simulink model "advanced_active_clamping"  (R2023b)
settings: Solver=ode1be  StartTime=0.0  StopTime=simlength  FixedStep=tc  RelTol=1e-3
values from neighbouring files (symbols this model uses):
  Rgate = 2.5    [init_model.m]
  Rgate_internal = 4    [init_model.m]
  t0_dpt = 5e-6    (= 5e-06)    [init_model.m]
  t1_dpt = t0_dpt + delta_time_first_pulse    (= 0.000105)    [init_model.m]
  t2_dpt = t1_dpt + deadtime    (= 0.000108)    [init_model.m]
  t3_dpt = t2_dpt + delta_time_discharge    (= 0.000128)    [init_model.m]
  t4_dpt = t3_dpt + deadtime    (= 0.000131)    [init_model.m]
  t5_dpt = t4_dpt + delta_time_second_pulse    (= 0.000166)    [init_model.m]
  t6_dpt = t5_dpt + deadtime    (= 0.000169)    [init_model.m]
  Vdc = 1400    [init_model.m]
  Vgate_h = 15    [init_model.m]
  Vgate_l = -7    [init_model.m]
libraries: fl_lib x55, nesl_utility x11, ee_lib x10, simulink x4
(part 3 of 3)

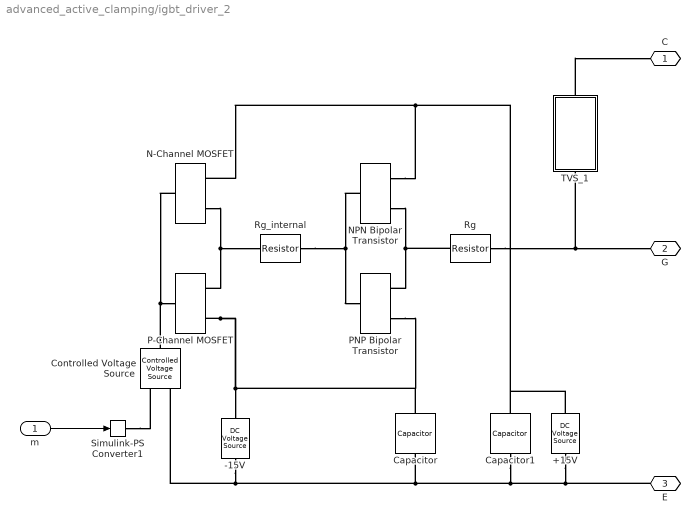
== system advanced_active_clamping/igbt_driver_2 ==
  m : Inport
  +15V : fl_lib/Electrical/Electrical Sources/DC Voltage Source  v0=15 V
  -15V : fl_lib/Electrical/Electrical Sources/DC Voltage Source  v0=-15 V
  Capacitor : fl_lib/Electrical/Electrical Elements/Capacitor  c=100e-9 F  r=1e-6 Ohm  g=0 1/Ohm  i_specify=off  i_priority=None  i=0 A  i_nominal_specify=off  i_nominal_unit=A  i_nominal_value=1  v_specify=off  v_priority=None  v=0 V  v_nominal_specify=off  v_nominal_unit=V  v_nominal_value=1  vc_specify=off  vc_priority=High  vc=0 V  vc_nominal_specify=off  vc_nominal_unit=V  vc_nominal_value=1
  Capacitor1 : fl_lib/Electrical/Electrical Elements/Capacitor  c=100e-9 F  r=1e-6 Ohm  g=0 1/Ohm  i_specify=off  i_priority=None  i=0 A  i_nominal_specify=off  i_nominal_unit=A  i_nominal_value=1  v_specify=off  v_priority=None  v=0 V  v_nominal_specify=off  v_nominal_unit=V  v_nominal_value=1  vc_specify=off  vc_priority=High  vc=0 V  vc_nominal_specify=off  vc_nominal_unit=V  vc_nominal_value=1
  Controlled Voltage Source : fl_lib/Electrical/Electrical Sources/Controlled Voltage Source
  N-Channel MOSFET : ee_lib/Semiconductors & Converters/N-Channel MOSFET  paramTerminal=ee.enum.mosfet.numberOfTerminals.three  parameterization=ee.enum.mosfet.parameterization.datasheet  Beta=5.0 A/V^2  Rds=0.025 Ohm  Id=100e-3 A  Vgs=10 V  Vth=1.7 V  Vth0=1.7 V  lam=0 1/V  gamma_vth=0.5 V^(1/2)  phib=0.5 V  Vth1=1.9071 V  Vbs1=-1 V  Vth2=2.066 V  Vbs2=-2 V  Tmeas=25 degC  Vgs_vec=[-1, -.5, 2, 3, 4, 5] V  Vds_vec=[0, 2, 4, 8, 12, 16, 20] V  Vbs_vec=[0, -4, -6, -12] V  T_vec=[25, 125] degC  Vth_vec=[.4, 1.2, 1.4, 1.45] V  Vth_mat=[.4, .35; 1.2, 1.15; 1.4, 1.35; 1.45, 1.4] V  Ids_mat=[0, 0, 0, 0, 0, 0, 0; 0, 0, 0, 0, 0, 0, 0; 0, .003, .0038, .0043, .0046, .0048, .0049; 0, .0055, .008, .009, .0095, .01, .0101; 0, .0115, .016, .018, .019, .0195, .02; 0, .0152, .0225, .0265, .028, .0295, .03] A  Ids_mat0=[0, 0, 0, 0, 0, 0, 0; 0, 0, 0, 0, 0, 0, 0; 0, .003, .0038, .0043, .0046, .0048, .0049; 0, .0055, .008, .009, .0095, .01, .0101; 0, .0115, .016, .018, .019, .0195, .02; 0, .0152, .0225, .0265, .028, .0295, .03] A  Ids_mat_3D=zeros(6, 7, 2) A  Ids_mat_3D0=zeros(6, 7, 2) A  IV_table_symmetry=ee.enum.mosfet.symmetricNIV.no  RS=0.0001 Ohm  RD=0.01 Ohm  RB=0.001 Ohm  C_param=ee.enum.mosfet.capacitanceParam.fixedciss  C_GS=270 pF  C_GD=80 pF  C_GB=0 pF  C_DS=0 pF  C_iss=350 pF  C_rss=80 pF  C_oss=0 pF  C_iss_vec=[720, 700, 590, 470, 390, 310] pF  C_rss_vec=[450, 400, 300, 190, 95, 55] pF  C_oss_vec=[900, 810, 690, 420, 270, 170] pF  C_GS_vec=[270, 300, 290, 280, 295, 255] pF  C_GD_vec=[450, 400, 300, 190, 95, 55] pF  C_GB_vec=[270, 300, 290, 280, 295, 255] pF  C_Vgs_vec=0 V  C_DS_vec=[450, 410, 390, 230, 175, 115] pF  C_Vds_vec=[.1, .3, 1, 3, 10, 30] V  V_GS_for_cap_data=0 V  charge_linearity_param=ee.enum.mosfet.cgdLinearity.constant  C_OX=200 pF  V_C_OX=-0.5 V  charge_linearity_param_vgb=ee.enum.mosfet.cgbLinearity.instantly  charge_linearity_param_with_vgb=ee.enum.mosfet.cgbLinearityWithSeparateCgb.instantly  Di_param=ee.enum.mosfet.diodeParam.no  IsDiode=1e-12 A  Vbi=0.6 V  n=1  Cj0Diode=0 pF  TT=50e-9 s  Tmeas_dio=25 degC  TableTypeNoT=ee.enum.mosfet.tableType.IfMat  TableType=ee.enum.diode.tableType.IfMat  IfVec=[.07, .12, .19, 1.75, 4.24, 7.32, 11.2] A  IfMat=[.07, .12, .19, 1.75, 4.24, 7.32, 11.2; .16, .3, .72, 2.14, 4.02, 6.35, 9.12] A  VfVecV=[.9, 1.15, 1.25, 1.5, 1.75, 2.17, 2.6, 2.85] V  VfMatV=[.9, 1.15, 1.25, 1.5, 1.75, 2.17, 2.6, 2.85; .58, .68, .75, 1.1, 1.38, 1.77, 2.27, 2.7] V  TjVec=[25, 125] degC  VfVec=[.5, .7, .9, 1.3, 1.7, 2.1, 2.5] V  IfVecV=[.1, .2, .5, 1, 2, 4, 7, 10] A  prmDatasheet=ee.enum.temperatureParameterization.none  prmEquCoeff=ee.enum.temperatureParameterization.none  dVth_dT=-6 mV/K  dVth0_dT=-6 mV/K  Rds_T2=0.037 Ohm  BEXDatasheet=-1.5  BEXEquCoeff=-1.5  etaisDatasheet=3  etaisEquCoeff=3  Tmeas2=125 degC  etaisTabulated=3  TdeviceDatasheet=25 degC  TdeviceEquCoeff=25 degC  TdeviceTabulated=25 degC  enable_faults=simscape.enum.onoff.off  fault_trigger=ee.enum.faults.faultTrigger.temporal  t_fault=inf s  max_permissible_Vgs=inf V  max_permissible_Vds=inf V  max_permissible_Vdb=inf V  max_permissible_Ids=inf A  t_fail_on_Ids=1 s  max_permissible_Idiode=inf A  t_fail_on_Idiode=1 s  max_permissible_dVdt=inf V/s  tau_fault=1e-3 s  fault_types=ee.enum.mosfet.faults.open  fault_types_4T=ee.enum.mosfet.faultsFourTerminals.open  RG_open=1e6 Ohm  RD_open=1000 Ohm  RS_open=1000 Ohm  RB_open=1000 Ohm  GDS_short=1000 1/Ohm  GDB_short=1000 1/Ohm  GSB_short=1000 1/Ohm  location_GOS=0  G_GOS=1000 1/Ohm  D_GOS=ee.enum.include.no  Is_GOS=0 A  Vbi_GOS=0.6 V  n_GOS=1  Cj0_GOS=0 pF  TT_GOS=50e-9 s  Beta_scale=100  dVth_faulted=0 V  lam_faulted=0 1/V  gamma_scale=100  dPhib_faulted=0 V  Vgs_vec_faulted=[-1, -.5, 2, 3, 4, 5] V  Vds_vec_faulted=[0, 2, 4, 8, 12, 16, 20] V  Vbs_vec_faulted=[0, -4, -6, -12] V  Vth_vec_faulted=[.4, 1.2, 1.4, 1.45] V  Vth_mat_faulted=[.4, .35; 1.2, 1.15; 1.4, 1.35; 1.45, 1.4] V  Ids_mat_faulted=[0, 0, 0, 0, 0, 0, 0; 0, 0, 0, 0, 0, 0, 0; 0, .003, .0038, .0043, .0046, .0048, .0049; 0, .0055, .008, .009, .0095, .01, .0101; 0, .0115, .016, .018, .019, .0195, .02; 0, .0152, .0225, .0265, .028, .0295, .03] A  Ids_mat0_faulted=[0, 0, 0, 0, 0, 0, 0; 0, 0, 0, 0, 0, 0, 0; 0, .003, .0038, .0043, .0046, .0048, .0049; 0, .0055, .008, .009, .0095, .01, .0101; 0, .0115, .016, .018, .019, .0195, .02; 0, .0152, .0225, .0265, .028, .0295, .03] A  Ids_mat_3D_faulted=zeros(6, 7, 2) A  Ids_mat_3D0_faulted=zeros(6, 7, 2) A  RS_faulted=0.0001 Ohm  RD_faulted=0.01 Ohm  RB_faulted=0.001 Ohm  IsDiode_faulted=0 A  Vbi_faulted=0.6 V  n_faulted=1  Cj0Diode_scale=100  TT_faulted=50e-9 s  IfVec_faulted=[.07, .12, .19, 1.75, 4.24, 7.32, 11.2] A  IfMat_faulted=[.07, .12, .19, 1.75, 4.24, 7.32, 11.2; .16, .3, .72, 2.14, 4.02, 6.35, 9.12] A  VfVecV_faulted=[.9, 1.15, 1.25, 1.5, 1.75, 2.17, 2.6, 2.85] V  VfMatV_faulted=[.9, 1.15, 1.25, 1.5, 1.75, 2.17, 2.6, 2.85; .58, .68, .75, 1.1, 1.38, 1.77, 2.27, 2.7] V  VfVec_faulted=[.5, .7, .9, 1.3, 1.7, 2.1, 2.5] V  IfVecV_faulted=[.1, .2, .5, 1, 2, 4, 7, 10] A  C_GS_scale=100  C_GD_scale=100  C_GB_scale=100  C_DS_scale=100  C_OX_scale=100  V_C_OX_faulted=-0.5 V  C_iss_vec_faulted=[720, 700, 590, 470, 390, 310] pF  C_rss_vec_faulted=[450, 400, 300, 190, 95, 55] pF  C_oss_vec_faulted=[900, 810, 690, 420, 270, 170] pF  C_GS_vec_faulted=[270, 300, 290, 280, 295, 255] pF  C_GD_vec_faulted=[450, 400, 300, 190, 95, 55] pF  C_GB_vec_faulted=[270, 300, 290, 280, 295, 255] pF  C_Vgs_vec_faulted=0 V  C_DS_vec_faulted=[450, 410, 390, 230, 175, 115] pF  C_Vds_vec_faulted=[.1, .3, 1, 3, 10, 30] V  V_GS_for_cap_data_faulted=0 V  i_g_specify=off  i_g_priority=None  i_g=0 A  i_g_nominal_specify=off  i_g_nominal_unit=A  i_g_nominal_value=1  i_d_specify=off  i_d_priority=None  i_d=0 A  i_d_nominal_specify=off  i_d_nominal_unit=A  i_d_nominal_value=1  i_b_specify=off  i_b_priority=None  i_b=0 A  i_b_nominal_specify=off  i_b_nominal_unit=A  i_b_nominal_value=1  voltage_gs_specify=off  voltage_gs_priority=None  voltage_gs=0 V  voltage_gs_nominal_specify=off  voltage_gs_nominal_unit=V  voltage_gs_nominal_value=1  voltage_ds_specify=off  voltage_ds_priority=None  voltage_ds=0 V  voltage_ds_nominal_specify=off  voltage_ds_nominal_unit=V  voltage_ds_nominal_value=1  voltage_bs_specify=off  voltage_bs_priority=None  voltage_bs=0 V  voltage_bs_nominal_specify=off  voltage_bs_nominal_unit=V  voltage_bs_nominal_value=1  v_Cgs_specify=off  v_Cgs_priority=High  v_Cgs=0 V  v_Cgs_nominal_specify=off  v_Cgs_nominal_unit=V  v_Cgs_nominal_value=1  v_Cds_specify=off  v_Cds_priority=High  v_Cds=0 V  v_Cds_nominal_specify=off  v_Cds_nominal_unit=V  v_Cds_nominal_value=1  v_Cbs_specify=off  v_Cbs_priority=High  v_Cbs=0 V  v_Cbs_nominal_specify=off  v_Cbs_nominal_unit=V  v_Cbs_nominal_value=1  faulted_specify=off  faulted_priority=None  faulted=0  faulted_nominal_specify=off  faulted_nominal_unit=1  faulted_nominal_value=1  thermal_network_parameterization=ee.enum.thermalNetworkTopology.junctionCase  Rth=[0, 10] K/W  Rth_Cauer=[1, 3, 10] K/W  Rth_Foster=[4, 6] K/W  thermal_mass_parameterization=ee.enum.thermalNetwork.timeconstant  thermal_mass=[0, 1] J/K  thermal_mass_Cauer=[.1, .3, 1] J/K  thermal_mass_Foster=[1.5, 3] J/K  thermal_time_constant=[0, 10] s  thermal_time_constant_Cauer=[1, 3, 10] s  thermal_time_constant_Foster=[6, 18] s  thermal_mass_initial_temperatures=[25, 25] degC  thermal_mass_initial_temperatures_Cauer=[25, 25, 25] degC  Tvec_initial_Foster=[25, 25, 25, 25] degC  max_permissible_temperature=inf K  t_fail_on_temperature=1 s  betaref=18 A/V^2  Vfbref=-1.1 V  gamma=3.5 V^(1/2)  phib2ref=1 V  thesatref=0.4 1/V  alpha=0  Vp=5e-2 V  thesrref=0 1/V  m=8  Tref=25 degC  Rsref=2e-3 Ohm  Rdref=0.17 Ohm  Rgref=8.4 Ohm  Rbref=2e-3 Ohm  Cox=1500 pF  Cgso=100 pF  Cgdo=14 pF  Isref=5.2e-13 A  Cj0=480 pF  Tprm=1  etabet=1.3  Stvfb=5e-4 V/K  Stphib=-8.5e-4 V/K  etasat=1.04  etasr=0.65  etar=0.95  etais=3  Tsim=25 degC  Ig_specify=off  Ig_priority=None  Ig=0 A  Ig_nominal_specify=off  Ig_nominal_unit=A  Ig_nominal_value=1  Ids_specify=off  Ids_priority=None  Ids=0 A  Ids_nominal_specify=off  Ids_nominal_unit=A  Ids_nominal_value=1  Ib_specify=off  Ib_priority=None  Ib=0 A  Ib_nominal_specify=off  Ib_nominal_unit=A  Ib_nominal_value=1  V_gs_specify=off  V_gs_priority=None  V_gs=0 V  V_gs_nominal_specify=off  V_gs_nominal_unit=V  V_gs_nominal_value=1  V_ds_specify=off  V_ds_priority=None  V_ds=0 V  V_ds_nominal_specify=off  V_ds_nominal_unit=V  V_ds_nominal_value=1  V_bs_specify=off  V_bs_priority=None  V_bs=0 V  V_bs_nominal_specify=off  V_bs_nominal_unit=V  V_bs_nominal_value=1  QGoverCox_specify=off  QGoverCox_priority=None  QGoverCox=0 V  QGoverCox_nominal_specify=off  QGoverCox_nominal_unit=V  QGoverCox_nominal_value=1  QDoverCox_specify=off  QDoverCox_priority=None  QDoverCox=0 V  QDoverCox_nominal_specify=off  QDoverCox_nominal_unit=V  QDoverCox_nominal_value=1  QBoverCox_specify=off  QBoverCox_priority=None  QBoverCox=0 V  QBoverCox_nominal_specify=off  QBoverCox_nominal_unit=V  QBoverCox_nominal_value=1  T0=[25, 25] degC  T0_Cauer=[25, 25, 25] degC
  NPN Bipolar Transistor : ee_lib/Semiconductors & Converters/NPN Bipolar Transistor  parameterization=1  BF=100  IS=1e-14 A  VAF=200 V  hfe=100  hoe=50e-6 1/Ohm  Ic_h=1 mA  Vce_h=5 V  V1=0.55 V  I1=0.5 mA  BR=1  Tmeas=25 degC  RC=0.01 Ohm  RE=1e-4 Ohm  RB=1 Ohm  C_BC=5 pF  C_BE=5 pF  TF=0 us  TR=0 us  prmDatasheet=1  prmEquCoeff=1  hfe_T2=125  XTB=0  V1_T2=0.45 V  I1_T2=0.5 mA  Tmeas2=125 degC  EG=1.11 eV  XTI=3  TdeviceDatasheet=25 degC  TdeviceEquCoeff=25 degC  ec=1  ib_specify=off  ib_priority=None  ib=0 A  ib_nominal_specify=off  ib_nominal_unit=A  ib_nominal_value=1  ic_specify=off  ic_priority=None  ic=0 A  ic_nominal_specify=off  ic_nominal_unit=A  ic_nominal_value=1  vce_specify=off  vce_priority=None  vce=0 V  vce_nominal_specify=off  vce_nominal_unit=V  vce_nominal_value=1  vbe_specify=off  vbe_priority=None  vbe=0 V  vbe_nominal_specify=off  vbe_nominal_unit=V  vbe_nominal_value=1  v_capacitor_bc_specify=off  v_capacitor_bc_priority=High  v_capacitor_bc=0 V  v_capacitor_bc_nominal_specify=off  v_capacitor_bc_nominal_unit=V  v_capacitor_bc_nominal_value=1  v_capacitor_be_specify=off  v_capacitor_be_priority=High  v_capacitor_be=0 V  v_capacitor_be_nominal_specify=off  v_capacitor_be_nominal_unit=V  v_capacitor_be_nominal_value=1  thermal_network_parameterization=ee.enum.thermalNetworkTopology.junctionCase  Rth=[0, 10] K/W  Rth_Cauer=[1, 3, 10] K/W  Rth_Foster=[4, 6] K/W  thermal_mass_parameterization=ee.enum.thermalNetwork.timeconstant  thermal_mass=[0, 1] J/K  thermal_mass_Cauer=[.1, .3, 1] J/K  thermal_mass_Foster=[1.5, 3] J/K  thermal_time_constant=[0, 10] s  thermal_time_constant_Cauer=[1, 3, 10] s  thermal_time_constant_Foster=[6, 18] s  thermal_mass_initial_temperatures=[25, 25] degC  thermal_mass_initial_temperatures_Cauer=[25, 25, 25] degC  Tvec_initial_Foster=[25, 25, 25, 25] degC
  P-Channel MOSFET : ee_lib/Semiconductors & Converters/P-Channel MOSFET  paramTerminal=ee.enum.mosfet.numberOfTerminals.three  parameterization=ee.enum.mosfet.parameterization.datasheet  Beta=2.0 A/V^2  Rds=0.025 Ohm  Id=-100e-3 A  Vgs=-4.5 V  Vth=-1.4 V  Vth0=-1.4 V  lam=0 1/V  gamma_vth=0.5 V^(1/2)  phib=0.5 V  Vth1=-1.6071 V  Vbs1=1 V  Vth2=-1.7660 V  Vbs2=2 V  Tmeas=25 degC  Vsg_vec=[-1, -.5, 2, 3, 4, 5] V  Vsd_vec=[0, 2, 4, 8, 12, 16, 20] V  Vsb_vec=[0, -4, -6, -12] V  T_vec=[25, 125] degC  Vth_vec=[-.4, -1.2, -1.4, -1.45] V  Vth_mat=[-.4, -.35; -1.2, -1.15; -1.4, -1.35; -1.45, -1.4] V  Isd_mat=[0, 0, 0, 0, 0, 0, 0; 0, 0, 0, 0, 0, 0, 0; 0, .003, .0038, .0043, .0046, .0048, .0049; 0, .0055, .008, .009, .0095, .01, .0101; 0, .0115, .016, .018, .019, .0195, .02; 0, .0152, .0225, .0265, .028, .0295, .03] A  Isd_mat0=[0, 0, 0, 0, 0, 0, 0; 0, 0, 0, 0, 0, 0, 0; 0, .003, .0038, .0043, .0046, .0048, .0049; 0, .0055, .008, .009, .0095, .01, .0101; 0, .0115, .016, .018, .019, .0195, .02; 0, .0152, .0225, .0265, .028, .0295, .03] A  Isd_mat_3D=zeros(6, 7, 2) A  Isd_mat_3D0=zeros(6, 7, 2) A  IV_table_symmetry=ee.enum.mosfet.symmetricPIV.no  RS=0.0001 Ohm  RD=0.01 Ohm  RB=0.001 Ohm  C_param=ee.enum.mosfet.capacitanceParam.fixedciss  C_GS=158 pF  C_GD=24 pF  C_GB=0 pF  C_DS=0 pF  C_iss=182 pF  C_rss=24 pF  C_oss=0 pF  C_iss_vec=[225, 210, 200, 185, 175, 170] pF  C_rss_vec=[75, 60, 50, 35, 25, 20] pF  C_oss_vec=[180, 160, 125, 80, 60, 45] pF  C_GS_vec=[150, 150, 150, 150, 150, 150] pF  C_GD_vec=[75, 60, 50, 35, 25, 20] pF  C_GB_vec=[450, 400, 300, 190, 95, 55] pF  C_Vsg_vec=0 V  C_DS_vec=[105, 100, 75, 45, 35, 25] pF  C_Vsd_vec=[.1, .3, 1, 3, 10, 30] V  V_GS_for_cap_data=0 V  charge_linearity_param=ee.enum.mosfet.cgdLinearity.constant  C_OX=200 pF  V_C_OX=0.5 V  charge_linearity_param_vgb=ee.enum.mosfet.cgbLinearity.instantly  charge_linearity_param_with_vgb=ee.enum.mosfet.cgbLinearityWithSeparateCgb.instantly  Di_param=ee.enum.mosfet.diodeParam.no  IsDiode=1e-12 A  Vbi=0.6 V  n=1  Cj0Diode=0 pF  TT=50e-9 s  Tmeas_dio=25 degC  TableTypeNoT=ee.enum.mosfet.tableType.IfMat  TableType=ee.enum.diode.tableType.IfMat  IfVec=[.07, .12, .19, 1.75, 4.24, 7.32, 11.2] A  IfMat=[.07, .12, .19, 1.75, 4.24, 7.32, 11.2; .16, .3, .72, 2.14, 4.02, 6.35, 9.12] A  VfVecV=[.9, 1.15, 1.25, 1.5, 1.75, 2.17, 2.6, 2.85] V  VfMatV=[.9, 1.15, 1.25, 1.5, 1.75, 2.17, 2.6, 2.85; .58, .68, .75, 1.1, 1.38, 1.77, 2.27, 2.7] V  TjVec=[25, 125] degC  VfVec=[.5, .7, .9, 1.3, 1.7, 2.1, 2.5] V  IfVecV=[.1, .2, .5, 1, 2, 4, 7, 10] A  prmDatasheet=ee.enum.temperatureParameterization.none  prmEquCoeff=ee.enum.temperatureParameterization.none  dVth_dT=2 mV/K  dVth0_dT=2 mV/K  Rds_T2=0.25 Ohm  BEXDatasheet=-1.5  BEXEquCoeff=-1.5  etaisDatasheet=3  etaisEquCoeff=3  Tmeas2=125 degC  etaisTabulated=3  TdeviceDatasheet=25 degC  TdeviceEquCoeff=25 degC  TdeviceTabulated=25 degC  enable_faults=simscape.enum.onoff.off  fault_trigger=ee.enum.faults.faultTrigger.temporal  t_fault=inf s  max_permissible_Vsg=inf V  max_permissible_Vsd=inf V  max_permissible_Vbd=inf V  max_permissible_Isd=inf A  t_fail_on_Isd=1 s  max_permissible_Idiode=inf A  t_fail_on_Idiode=1 s  max_permissible_dVdt=inf V/s  tau_fault=1e-3 s  fault_types=ee.enum.mosfet.faults.open  fault_types_4T=ee.enum.mosfet.faultsFourTerminals.open  RG_open=1e6 Ohm  RD_open=1000 Ohm  RS_open=1000 Ohm  RB_open=1000 Ohm  GDS_short=1000 1/Ohm  GDB_short=1000 1/Ohm  GSB_short=1000 1/Ohm  location_GOS=0  G_GOS=1000 1/Ohm  D_GOS=ee.enum.include.no  Is_GOS=0 A  Vbi_GOS=0.6 V  n_GOS=1  Cj0_GOS=0 pF  TT_GOS=50e-9 s  Beta_scale=100  dVth_faulted=0 V  lam_faulted=0 1/V  gamma_scale=100  dPhib_faulted=0 V  Vsg_vec_faulted=[-1, -.5, 2, 3, 4, 5] V  Vsd_vec_faulted=[0, 2, 4, 8, 12, 16, 20] V  Vsb_vec_faulted=[0, -4, -6, -12] V  Vth_vec_faulted=[-.4, -1.2, -1.4, -1.45] V  Vth_mat_faulted=[-.4, -.35; -1.2, -1.15; -1.4, -1.35; -1.45, -1.4] V  Isd_mat_faulted=[0, 0, 0, 0, 0, 0, 0; 0, 0, 0, 0, 0, 0, 0; 0, .003, .0038, .0043, .0046, .0048, .0049; 0, .0055, .008, .009, .0095, .01, .0101; 0, .0115, .016, .018, .019, .0195, .02; 0, .0152, .0225, .0265, .028, .0295, .03] A  Isd_mat0_faulted=[0, 0, 0, 0, 0, 0, 0; 0, 0, 0, 0, 0, 0, 0; 0, .003, .0038, .0043, .0046, .0048, .0049; 0, .0055, .008, .009, .0095, .01, .0101; 0, .0115, .016, .018, .019, .0195, .02; 0, .0152, .0225, .0265, .028, .0295, .03] A  Isd_mat_3D_faulted=zeros(6, 7, 2) A  Isd_mat_3D0_faulted=zeros(6, 7, 2) A  RS_faulted=0.0001 Ohm  RD_faulted=0.01 Ohm  RB_faulted=0.001 Ohm  IsDiode_faulted=0 A  Vbi_faulted=0.6 V  n_faulted=1  Cj0Diode_scale=100  TT_faulted=50e-9 s  IfVec_faulted=[.07, .12, .19, 1.75, 4.24, 7.32, 11.2] A  IfMat_faulted=[.07, .12, .19, 1.75, 4.24, 7.32, 11.2; .16, .3, .72, 2.14, 4.02, 6.35, 9.12] A  VfVecV_faulted=[.9, 1.15, 1.25, 1.5, 1.75, 2.17, 2.6, 2.85] V  VfMatV_faulted=[.9, 1.15, 1.25, 1.5, 1.75, 2.17, 2.6, 2.85; .58, .68, .75, 1.1, 1.38, 1.77, 2.27, 2.7] V  VfVec_faulted=[.5, .7, .9, 1.3, 1.7, 2.1, 2.5] V  IfVecV_faulted=[.1, .2, .5, 1, 2, 4, 7, 10] A  C_GS_scale=100  C_GD_scale=100  C_GB_scale=100  C_DS_scale=100  C_OX_scale=100  V_C_OX_faulted=0.5 V  C_iss_vec_faulted=[720, 700, 590, 470, 390, 310] pF  C_rss_vec_faulted=[450, 400, 300, 190, 95, 55] pF  C_oss_vec_faulted=[900, 810, 690, 420, 270, 170] pF  C_GS_vec_faulted=[270, 300, 290, 280, 295, 255] pF  C_GD_vec_faulted=[450, 400, 300, 190, 95, 55] pF  C_GB_vec_faulted=[270, 300, 290, 280, 295, 255] pF  C_Vsg_vec_faulted=0 V  C_DS_vec_faulted=[450, 410, 390, 230, 175, 115] pF  C_Vsd_vec_faulted=[.1, .3, 1, 3, 10, 30] V  V_GS_for_cap_data_faulted=0 V  i_g_specify=off  i_g_priority=None  i_g=0 A  i_g_nominal_specify=off  i_g_nominal_unit=A  i_g_nominal_value=1  i_d_specify=off  i_d_priority=None  i_d=0 A  i_d_nominal_specify=off  i_d_nominal_unit=A  i_d_nominal_value=1  i_b_specify=off  i_b_priority=None  i_b=0 A  i_b_nominal_specify=off  i_b_nominal_unit=A  i_b_nominal_value=1  voltage_gs_specify=off  voltage_gs_priority=None  voltage_gs=0 V  voltage_gs_nominal_specify=off  voltage_gs_nominal_unit=V  voltage_gs_nominal_value=1  voltage_ds_specify=off  voltage_ds_priority=None  voltage_ds=0 V  voltage_ds_nominal_specify=off  voltage_ds_nominal_unit=V  voltage_ds_nominal_value=1  voltage_bs_specify=off  voltage_bs_priority=None  voltage_bs=0 V  voltage_bs_nominal_specify=off  voltage_bs_nominal_unit=V  voltage_bs_nominal_value=1  v_Cgs_specify=off  v_Cgs_priority=High  v_Cgs=0 V  v_Cgs_nominal_specify=off  v_Cgs_nominal_unit=V  v_Cgs_nominal_value=1  v_Cds_specify=off  v_Cds_priority=High  v_Cds=0 V  v_Cds_nominal_specify=off  v_Cds_nominal_unit=V  v_Cds_nominal_value=1  v_Cbs_specify=off  v_Cbs_priority=High  v_Cbs=0 V  v_Cbs_nominal_specify=off  v_Cbs_nominal_unit=V  v_Cbs_nominal_value=1  faulted_specify=off  faulted_priority=None  faulted=0  faulted_nominal_specify=off  faulted_nominal_unit=1  faulted_nominal_value=1  thermal_network_parameterization=ee.enum.thermalNetworkTopology.junctionCase  Rth=[0, 10] K/W  Rth_Cauer=[1, 3, 10] K/W  Rth_Foster=[4, 6] K/W  thermal_mass_parameterization=ee.enum.thermalNetwork.timeconstant  thermal_mass=[0, 1] J/K  thermal_mass_Cauer=[.1, .3, 1] J/K  thermal_mass_Foster=[1.5, 3] J/K  thermal_time_constant=[0, 10] s  thermal_time_constant_Cauer=[1, 3, 10] s  thermal_time_constant_Foster=[6, 18] s  thermal_mass_initial_temperatures=[25, 25] degC  thermal_mass_initial_temperatures_Cauer=[25, 25, 25] degC  Tvec_initial_Foster=[25, 25, 25, 25] degC  max_permissible_temperature=inf K  t_fail_on_temperature=1 s  betaref=18 A/V^2  Vfbref=-1.1 V  gamma=3.5 V^(1/2)  phib2ref=1 V  thesatref=0.4 1/V  alpha=0  Vp=5e-2 V  thesrref=0 1/V  m=8  Tref=25 degC  Rsref=2e-3 Ohm  Rdref=0.17 Ohm  Rgref=8.4 Ohm  Rbref=2e-3 Ohm  Cox=1500 pF  Cgso=100 pF  Cgdo=14 pF  Isref=5.2e-13 A  Cj0=480 pF  Tprm=1  etabet=1.3  Stvfb=5e-4 V/K  Stphib=-8.5e-4 V/K  etasat=1.04  etasr=0.65  etar=0.95  etais=3  Tsim=25 degC  Ig_specify=off  Ig_priority=None  Ig=0 A  Ig_nominal_specify=off  Ig_nominal_unit=A  Ig_nominal_value=1  Ids_specify=off  Ids_priority=None  Ids=0 A  Ids_nominal_specify=off  Ids_nominal_unit=A  Ids_nominal_value=1  Ib_specify=off  Ib_priority=None  Ib=0 A  Ib_nominal_specify=off  Ib_nominal_unit=A  Ib_nominal_value=1  V_gs_specify=off  V_gs_priority=None  V_gs=0 V  V_gs_nominal_specify=off  V_gs_nominal_unit=V  V_gs_nominal_value=1  V_ds_specify=off  V_ds_priority=None  V_ds=0 V  V_ds_nominal_specify=off  V_ds_nominal_unit=V  V_ds_nominal_value=1  V_bs_specify=off  V_bs_priority=None  V_bs=0 V  V_bs_nominal_specify=off  V_bs_nominal_unit=V  V_bs_nominal_value=1  QGoverCox_specify=off  QGoverCox_priority=None  QGoverCox=0 V  QGoverCox_nominal_specify=off  QGoverCox_nominal_unit=V  QGoverCox_nominal_value=1  QDoverCox_specify=off  QDoverCox_priority=None  QDoverCox=0 V  QDoverCox_nominal_specify=off  QDoverCox_nominal_unit=V  QDoverCox_nominal_value=1  QBoverCox_specify=off  QBoverCox_priority=None  QBoverCox=0 V  QBoverCox_nominal_specify=off  QBoverCox_nominal_unit=V  QBoverCox_nominal_value=1  T0=[25, 25] degC  T0_Cauer=[25, 25, 25] degC
      settings: InternalSimscapePortConfiguration="{\"Bottom\":[],\"Left\":[{\"id\":\"G\",\"label\":\"\",\"type\":\"foundation.electrical.electrical\"}],\"Right\":[{\"id\":\"S\",\"label\":\"s\",\"type\":\"foundation.electrical.electrical\"},{\"id\":\"D\",\"label\":\"d\",\"type\":\"foundation.electrical.electrical\"}],\"Top\":[]}"
  PNP Bipolar Transistor : ee_lib/Semiconductors & Converters/PNP Bipolar Transistor  parameterization=1  BF=100  IS=1e-14 A  VAF=200 V  hfe=100  hoe=50e-6 1/Ohm  Ic_h=-1 mA  Vce_h=-5 V  V1=-0.55 V  I1=-0.5 mA  BR=1  Tmeas=25 degC  RC=0.01 Ohm  RE=1e-4 Ohm  RB=1 Ohm  C_BC=5 pF  C_BE=5 pF  TF=0 us  TR=0 us  prmDatasheet=1  prmEquCoeff=1  hfe_T2=125  XTB=0  V1_T2=-0.45 V  I1_T2=-0.5 mA  Tmeas2=125 degC  EG=1.11 eV  XTI=3  TdeviceDatasheet=25 degC  TdeviceEquCoeff=25 degC  ec=1  ib_specify=off  ib_priority=None  ib=0 A  ib_nominal_specify=off  ib_nominal_unit=A  ib_nominal_value=1  ic_specify=off  ic_priority=None  ic=0 A  ic_nominal_specify=off  ic_nominal_unit=A  ic_nominal_value=1  vce_specify=off  vce_priority=None  vce=0 V  vce_nominal_specify=off  vce_nominal_unit=V  vce_nominal_value=1  vbe_specify=off  vbe_priority=None  vbe=0 V  vbe_nominal_specify=off  vbe_nominal_unit=V  vbe_nominal_value=1  v_capacitor_bc_specify=off  v_capacitor_bc_priority=High  v_capacitor_bc=0 V  v_capacitor_bc_nominal_specify=off  v_capacitor_bc_nominal_unit=V  v_capacitor_bc_nominal_value=1  v_capacitor_be_specify=off  v_capacitor_be_priority=High  v_capacitor_be=0 V  v_capacitor_be_nominal_specify=off  v_capacitor_be_nominal_unit=V  v_capacitor_be_nominal_value=1  thermal_network_parameterization=ee.enum.thermalNetworkTopology.junctionCase  Rth=[0, 10] K/W  Rth_Cauer=[1, 3, 10] K/W  Rth_Foster=[4, 6] K/W  thermal_mass_parameterization=ee.enum.thermalNetwork.timeconstant  thermal_mass=[0, 1] J/K  thermal_mass_Cauer=[.1, .3, 1] J/K  thermal_mass_Foster=[1.5, 3] J/K  thermal_time_constant=[0, 10] s  thermal_time_constant_Cauer=[1, 3, 10] s  thermal_time_constant_Foster=[6, 18] s  thermal_mass_initial_temperatures=[25, 25] degC  thermal_mass_initial_temperatures_Cauer=[25, 25, 25] degC  Tvec_initial_Foster=[25, 25, 25, 25] degC
      settings: InternalSimscapePortConfiguration="{\"Bottom\":[],\"Left\":[{\"id\":\"B\",\"label\":\"\",\"type\":\"foundation.electrical.electrical\"}],\"Right\":[{\"id\":\"n\",\"label\":\"\",\"type\":\"foundation.electrical.electrical\"},{\"id\":\"p\",\"label\":\"\",\"type\":\"foundation.electrical.electrical\"}],\"Top\":[]}"
  Rg : fl_lib/Electrical/Electrical Elements/Resistor  R=Rgate Ohm  i_specify=off  i_priority=None  i=0 A  i_nominal_specify=off  i_nominal_unit=A  i_nominal_value=1  v_specify=off  v_priority=None  v=0 V  v_nominal_specify=off  v_nominal_unit=V  v_nominal_value=1
  Rg_internal : fl_lib/Electrical/Electrical Elements/Resistor  R=Rgate_internal Ohm  i_specify=off  i_priority=None  i=0 A  i_nominal_specify=off  i_nominal_unit=A  i_nominal_value=1  v_specify=off  v_priority=None  v=0 V  v_nominal_specify=off  v_nominal_unit=V  v_nominal_value=1
  Simulink-PS Converter1 : nesl_utility/Simulink-PS Converter  PhysicalDomain=network_engine_domain  SubClassName=ps_input  LeftPortType=input  RightPortType=output  PseudoPeriodic=off  Frequencies=[]  NoiseDistribution=none  NoiseParameters=[]  Unit=V  AffineConversion=off  FilteringAndDerivatives=provide  SimscapeFilterOrder=1  InputFilterTimeConstant=0.001  UdotUserProvided=0
  TVS_1 : Subsystem
      settings: PortSchema="{\"entries\":[{\"content\":{\"sides\":[{\"content\":{},\"type\":\"ConnectorPlacement.EquallySpacedRectSide\",\"uuid\":\"ceae994e-5469-4611-a745-44e177716c46\"},{\"content\":{\"side\":\"RIGHT\"},\"type\":\"ConnectorPlacement.EquallySpacedRectSide\",\"uuid\":\"7376ca02-a2b7-4760-b24d-ff5396d14cb7\"},{\"content\":{\"connectorIds\":[\"LConn1\"],\"side\":\"TOP\"},\"type\":\"ConnectorPlacement.EquallySpacedRectSide\",\"uuid\":\"e5d89c91-02bc-49cf-874d-f21a3fc48061\"},{\"content\":{\"connectorIds\":[\"RConn1\"],\"side\":\"BOTTOM\"},\"type\":\"ConnectorPlacement.EquallySpacedRectSide\",\"uuid\":\"df392675-ed98-4ecb-8641-1f46308e0272\"}]},\"type\":\"ConnectorPlacement.EquallySpacedConnector\",\"uuid\":\"073a1f26-4655-4d3d-9bad-7eb8f66fb459\"}],\"packageUris\":[\"http://schema.mathworks.com/mf0/Connector/R2020b\"],\"version\":\"1.0\"}"
  C : PMIOPort  Side=Left
  G : PMIOPort  Port=2  Side=Right
  E : PMIOPort  Port=3  Side=Right
  wires:
  m/1 -> Simulink-PS Converter1/1
  connections:
  Rg/LConn1 -- TVS_1/RConn1 -- G/RConn1
  TVS_1/LConn1 -- C/RConn1
  N-Channel MOSFET/RConn2 -- P-Channel MOSFET/RConn1 -- Rg_internal/RConn1
  N-Channel MOSFET/LConn1 -- Controlled Voltage Source/LConn1 -- P-Channel MOSFET/LConn1
  +15V/LConn1 -- Capacitor1/LConn1 -- NPN Bipolar Transistor/RConn1 -- N-Channel MOSFET/RConn1
  P-Channel MOSFET/RConn2 -- Capacitor/LConn1 -- PNP Bipolar Transistor/RConn2 -- -15V/LConn1
  Simulink-PS Converter1/RConn1 -- Controlled Voltage Source/RConn1
  E/RConn1 -- +15V/RConn1 -- -15V/RConn1 -- Controlled Voltage Source/RConn2 -- Capacitor/RConn1 -- Capacitor1/RConn1
  NPN Bipolar Transistor/RConn2 -- Rg/RConn1 -- PNP Bipolar Transistor/RConn1
  NPN Bipolar Transistor/LConn1 -- Rg_internal/LConn1 -- PNP Bipolar Transistor/LConn1

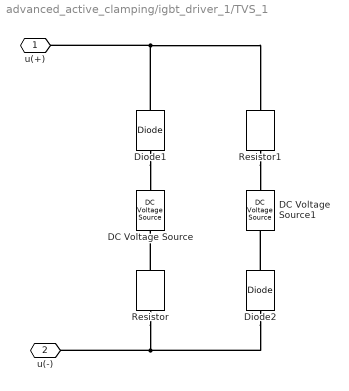
== system advanced_active_clamping/igbt_driver_1/TVS_1 ==
  DC Voltage Source : fl_lib/Electrical/Electrical Sources/DC Voltage Source  v0=1340 V
  DC Voltage Source1 : fl_lib/Electrical/Electrical Sources/DC Voltage Source  v0=1340 V
  Diode1 : fl_lib/Electrical/Electrical Elements/Diode  Vf=0.6 V  Ron=0.3 Ohm  Goff=1e-8 1/Ohm  i_specify=off  i_priority=None  i=0 A  i_nominal_specify=off  i_nominal_unit=A  i_nominal_value=1  v_specify=off  v_priority=None  v=0 V  v_nominal_specify=off  v_nominal_unit=V  v_nominal_value=1
  Diode2 : fl_lib/Electrical/Electrical Elements/Diode  Vf=0.6 V  Ron=0.3 Ohm  Goff=1e-8 1/Ohm  i_specify=off  i_priority=None  i=0 A  i_nominal_specify=off  i_nominal_unit=A  i_nominal_value=1  v_specify=off  v_priority=None  v=0 V  v_nominal_specify=off  v_nominal_unit=V  v_nominal_value=1
  Resistor : fl_lib/Electrical/Electrical Elements/Resistor  R=1 Ohm  i_specify=off  i_priority=None  i=0 A  i_nominal_specify=off  i_nominal_unit=A  i_nominal_value=1  v_specify=off  v_priority=None  v=0 V  v_nominal_specify=off  v_nominal_unit=V  v_nominal_value=1
  Resistor1 : fl_lib/Electrical/Electrical Elements/Resistor  R=1 Ohm  i_specify=off  i_priority=None  i=0 A  i_nominal_specify=off  i_nominal_unit=A  i_nominal_value=1  v_specify=off  v_priority=None  v=0 V  v_nominal_specify=off  v_nominal_unit=V  v_nominal_value=1
  u(+) : PMIOPort  Side=Left
  u(-) : PMIOPort  Port=2  Side=Right
  connections:
  Resistor/RConn1 -- Diode2/LConn1 -- u(-)/RConn1
  Resistor/LConn1 -- DC Voltage Source/RConn1
  Diode1/RConn1 -- DC Voltage Source/LConn1
  Diode1/LConn1 -- Resistor1/RConn1 -- u(+)/RConn1
  Diode2/RConn1 -- DC Voltage Source1/LConn1
  Resistor1/LConn1 -- DC Voltage Source1/RConn1

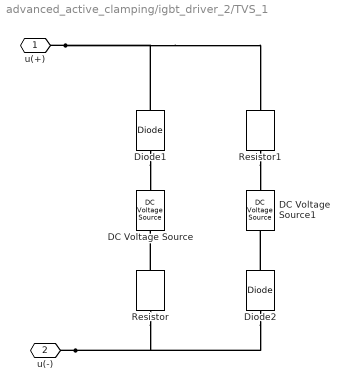
== system advanced_active_clamping/igbt_driver_2/TVS_1 ==
  DC Voltage Source : fl_lib/Electrical/Electrical Sources/DC Voltage Source  v0=1340 V
  DC Voltage Source1 : fl_lib/Electrical/Electrical Sources/DC Voltage Source  v0=1340 V
  Diode1 : fl_lib/Electrical/Electrical Elements/Diode  Vf=0.6 V  Ron=0.3 Ohm  Goff=1e-8 1/Ohm  i_specify=off  i_priority=None  i=0 A  i_nominal_specify=off  i_nominal_unit=A  i_nominal_value=1  v_specify=off  v_priority=None  v=0 V  v_nominal_specify=off  v_nominal_unit=V  v_nominal_value=1
  Diode2 : fl_lib/Electrical/Electrical Elements/Diode  Vf=0.6 V  Ron=0.3 Ohm  Goff=1e-8 1/Ohm  i_specify=off  i_priority=None  i=0 A  i_nominal_specify=off  i_nominal_unit=A  i_nominal_value=1  v_specify=off  v_priority=None  v=0 V  v_nominal_specify=off  v_nominal_unit=V  v_nominal_value=1
  Resistor : fl_lib/Electrical/Electrical Elements/Resistor  R=1 Ohm  i_specify=off  i_priority=None  i=0 A  i_nominal_specify=off  i_nominal_unit=A  i_nominal_value=1  v_specify=off  v_priority=None  v=0 V  v_nominal_specify=off  v_nominal_unit=V  v_nominal_value=1
  Resistor1 : fl_lib/Electrical/Electrical Elements/Resistor  R=1 Ohm  i_specify=off  i_priority=None  i=0 A  i_nominal_specify=off  i_nominal_unit=A  i_nominal_value=1  v_specify=off  v_priority=None  v=0 V  v_nominal_specify=off  v_nominal_unit=V  v_nominal_value=1
  u(+) : PMIOPort  Side=Left
  u(-) : PMIOPort  Port=2  Side=Right
  connections:
  Resistor1/LConn1 -- DC Voltage Source1/RConn1
  Diode2/RConn1 -- DC Voltage Source1/LConn1
  u(+)/RConn1 -- Resistor1/RConn1 -- Diode1/LConn1
  Diode1/RConn1 -- DC Voltage Source/LConn1
  Resistor/LConn1 -- DC Voltage Source/RConn1
  u(-)/RConn1 -- Diode2/LConn1 -- Resistor/RConn1
